simulink model "ssc_aircraft_elec_hybrid"  (R2025a)
settings: Solver=ode23t  StartTime=0.0  StopTime=FlightProfileLength  RelTol=1e-3  AbsTol=1e-3  EnableMultiTasking=on
PreLoadFcn:
  | ssc_aircraft_elec_default_params
PostLoadFcn:
  | warning('off','physmod:common:gl:sli:rtp:InvalidNonValueReference')
  | warning off Simulink:Engine:SortDiscontinuityInAlgLoop
model workspace (MATLAB code in the model file):
  | v0                 = 0; % Initial vehicle speed
  | wheel_radius = 0.15; % Wheel radius
  | k                   = 1e-2; % Motor losses (W/(N*M)^2)
  | t_torque        = 0.02; % Electric motor time constant
  | rpm0             = 2000; % Engine initial speed demand
undefined symbols (not defined in the file): Based, engine_ref_speed, gen_torque_demand, Height, motor_ref_speed
libraries: fl_lib x53, nesl_utility x31, ee_lib x9, ssc_aircraft_elec_lib x2, batteryecm_lib x1, simulink x1, sdl_lib x1, SimscapeFluids_lib x1
(part 2 of 2)

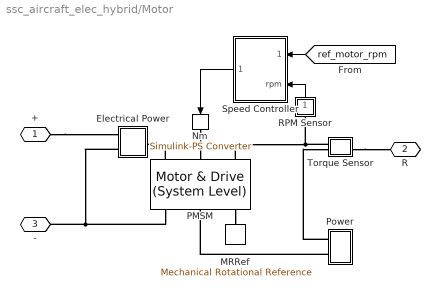
== system ssc_aircraft_elec_hybrid/Motor ==
  Electrical Power : Subsystem
  MRRef : fl_lib/Mechanical/Rotational Elements/Mechanical Rotational Reference
  Nm : nesl_utility/Simulink-PS Converter  PhysicalDomain=network_engine_domain  SubClassName=ps_input  LeftPortType=input  RightPortType=output  PseudoPeriodic=off  Frequencies=[]  NoiseDistribution=none  NoiseParameters=[]  Unit=N*m  AffineConversion=off  FilteringAndDerivatives=zero  SimscapeFilterOrder=1  InputFilterTimeConstant=.001  UdotUserProvided=1
  PMSM : ee_lib/Electromechanical/Motor & Drive (System Level)  torque_speed_param=1  overtorque_param=ee.enum.electromech.overtorque.no  T_t=[ 0.9 0.8 0.7 0 ]*500 N*m  T_t_intermittent=[.36, .32, .28, 0] N*m  T_t_2D=[.09, .09, .09; .08, .08, .08; .07, .07, .07; 0, 0, 0] N*m  T_t_intermittent_2D=[.36, .36, .36; .32, .32, .32; .28, .28, .28; 0, 0, 0] N*m  w_t=[ 0 3.75e+3 7.5e+3 8e+3 ] rpm  vdc_t=[6, 12, 24] V  torque_max=0.1 N*m  power_max=30 W  torque_max_intermittent=0.4 N*m  power_max_intermittent=120 W  time_overtorque=30 s  time_recover=60 s  Tc=0.02 s  EnableSwitch=simscape.enum.onoff.off  losses_param=1  eff=95  w_eff=3.75e+3 rpm  T_eff=400 N*m  Piron=0 W  Pbase=0 W  w_eff_vec=[-8000 -4000 0 4000 8000] rpm  T_eff_vec=[0 0.03 0.06 0.09] N*m  v_eff_vec=[100, 250, 400] V  losses_mat=[1.49 1.67 2.21 3.10; 0.42 0.69 1.14 2.03; 0.06 0.24 0.78 1.68; 0.42 0.69 1.14 2.03; 1.49 1.67 2.21 3.10] W  efficiency_mat=[95 95 95 95; 95 95 95 95; 95 95 95 95; 95 95 95 95; 95 95 95 95]  losses_mat_3D=ones(5, 4, 3) W  efficiency_mat_3D=95 * ones(5, 4, 3)  Res=0 Ohm  J=0 kg*m^2  lam=1e-5 N*m/(rad/s)  speed0=2000 rpm  faulted_specify=off  faulted_priority=None  faulted=0  faulted_nominal_specify=off  faulted_nominal_value=1  faulted_nominal_unit=1  isSwitchedOff_specify=off  isSwitchedOff_priority=None  isSwitchedOff=0  isSwitchedOff_nominal_specify=off  isSwitchedOff_nominal_value=1  isSwitchedOff_nominal_unit=1  torqueLimitContinuous_specify=off  torqueLimitContinuous_priority=None  torqueLimitContinuous=0 N*m  torqueLimitContinuous_nominal_specify=off  torqueLimitContinuous_nominal_value=1  torqueLimitContinuous_nominal_unit=N*m  alpha=3.93e-3 1/K  Tmeas=25 degC  Tmeas2=125 degC  losses_mat_T2=[1.49, 1.74, 2.49, 3.74; .42, .67, 1.42, 2.67; .06, .31, 1.06, 2.31; .42, .67, 1.42, 2.67; 1.49, 1.74, 2.49, 3.74] W  efficiency_mat_T2=[95, 95, 95, 95; 95, 95, 95, 95; 95, 95, 95, 95; 95, 95, 95, 95; 95, 95, 95, 95]  losses_mat_3D_T2=ones(5, 4, 3) W  efficiency_mat_3D_T2=95 * ones(5, 4, 3)  thermal_mass=100 J/K  initial_temperature=25 degC
  Power : Subsystem
  RPM Sensor : Subsystem
      mask Display: disp('w')
  Speed Controller : Subsystem
  Torque Sensor : Subsystem
      mask Display: disp('trq');
  + : PMIOPort  Side=Right
  R : PMIOPort  Port=2  Side=Left
  - : PMIOPort  Port=3  Side=Right
  wires:
  Speed Controller/1(T_ref) -> Nm/1
  [ref_motor_rpm] -> Speed Controller/1(rpm_ref)
  RPM Sensor/1(rpm) -> Speed Controller/2(rpm)
  connections:
  Power/RConn2 -- PMSM/RConn2
  Torque Sensor/RConn1 -- R/RConn1
  Nm/RConn1 -- PMSM/LConn2
  PMSM/LConn3 -- RPM Sensor/LConn1 -- Torque Sensor/LConn1
  Electrical Power/LConn2 -- -/RConn1 -- PMSM/RConn1
  PMSM/LConn1 -- Electrical Power/RConn1
  PMSM/RConn3 -- MRRef/LConn1
  +/RConn1 -- Electrical Power/LConn1
  Power/RConn1 -- Torque Sensor/LConn2

== system ssc_aircraft_elec_hybrid/Routing ==
  M : Inport
  E : Inport  Port=2
  G : Inport  Port=3
  tag scope: ref_engine_speed=global, ref_generator_torque=global, ref_motor_rpm=global
  wires:
  M/1 -> [ref_motor_rpm]  "Ref Motor RPM"
  G/1 -> [ref_generator_torque]
  E/1 -> [ref_engine_speed]

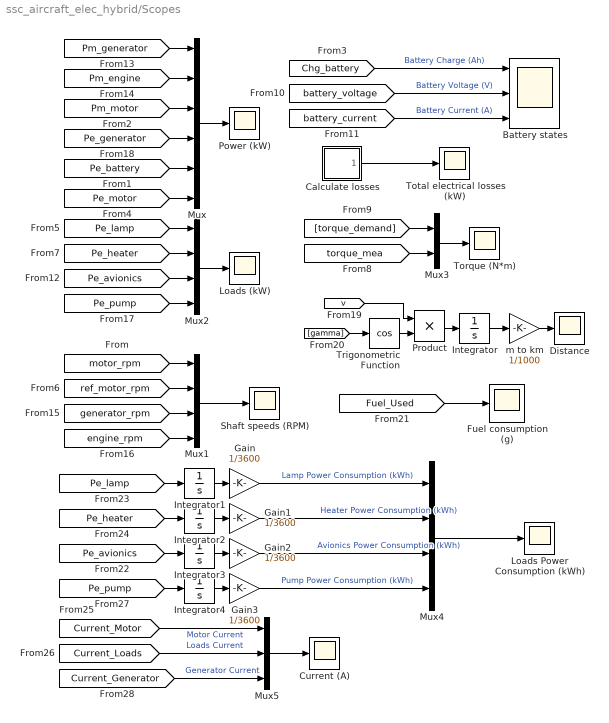
== system ssc_aircraft_elec_hybrid/Scopes ==
  Battery states : Scope  NumInputPorts=3
      settings: ActiveDisplayYMinimum=10  ActiveDisplayYMaximum=110  DataLoggingVariableName=HybridBatteryScopeData
  Calculate losses : Subsystem
  Current (A) : Scope
      settings: TimeSpan=20  ActiveDisplayYMinimum=-113.26291  ActiveDisplayYMaximum=160.64128  DataLoggingMaxPoints=50000  DataLoggingVariableName=HybridCurrentData
  Distance : Scope
      settings: ActiveDisplayYMinimum=-12.7724  ActiveDisplayYMaximum=114.9516  DataLoggingVariableName=Distance  DataLoggingSaveFormat=Array
  Fuel consumption (g) : Scope
      settings: TimeSpan=20  ActiveDisplayYMinimum=-191.16919  ActiveDisplayYMaximum=1720.52275  DataLoggingMaxPoints=50000
  Gain{,1..3} (4 alike) : Gain  Gain=1/3600
  Integrator{,1..4} (5 alike) : Integrator
  Loads (kW) : Scope
      settings: TimeSpan=20  ActiveDisplayYMinimum=-0.2683  ActiveDisplayYMaximum=2.41473  DataLoggingMaxPoints=50000
  Loads Power Consumption (kWh) : Scope
      settings: TimeSpan=20  ActiveDisplayYMinimum=-0.06156  ActiveDisplayYMaximum=0.55406  DataLoggingMaxPoints=50000  DataLoggingVariableName=HybridLoadPowerConsumptionData
  Mux : Mux  Inputs=6
  Mux1 : Mux
  Mux2 : Mux
  Mux3 : Mux  Inputs=2
  Mux4 : Mux
  Mux5 : Mux  Inputs=3
  Power (kW) : Scope
      settings: TimeSpan=20  ActiveDisplayYMinimum=-16.03345  ActiveDisplayYMaximum=35.31999  DataLoggingMaxPoints=50000  DataLoggingVariableName=ScopeData8
  Product : Product
  Shaft speeds (RPM) : Scope
      settings: ActiveDisplayYMinimum=1473.13164  ActiveDisplayYMaximum=2062.04487  DataLoggingMaxPoints=50000
  Torque (N*m) : Scope
      settings: TimeSpan=20  ActiveDisplayYMinimum=-49.62729  ActiveDisplayYMaximum=446.62471  DataLoggingMaxPoints=50000
  Total electrical losses (kW) : Scope
      settings: TimeSpan=20  ActiveDisplayYMinimum=1.3595  ActiveDisplayYMaximum=5.38899  DataLoggingVariableName=ScopeData3
  Trigonometric Function : Trigonometry  Operator=cos
  m to km : Gain  Gain=1/1000
  wires:
  [Chg_battery] -> Battery states/1  "Battery Charge (Ah)"
  Calculate losses/1(Ploss) -> Total electrical losses (kW)/1
  [Pe_battery] -> Mux/5
  [motor_rpm] -> Mux1/1
  Mux1/1 -> Shaft speeds (RPM)/1
  Mux/1 -> Power (kW)/1
  Mux2/1 -> Loads (kW)/1
  [Pe_motor] -> Mux/6
  [Pm_motor] -> Mux/3
  [ref_motor_rpm] -> Mux1/2
  Mux3/1 -> Torque (N*m)/1
  [torque_demand] -> Mux3/1
  [torque_mea] -> Mux3/2
  [battery_voltage] -> Battery states/2  "Battery Voltage (V)"
  [battery_current] -> Battery states/3  "Battery Current (A)"
  [Pe_avionics] -> Mux2/3
  [Pe_lamp] -> Mux2/1
  [Pe_heater] -> Mux2/2
  [Pm_generator] -> Mux/1
  [Pm_engine] -> Mux/2
  [generator_rpm] -> Mux1/3
  [engine_rpm] -> Mux1/4
  [Pe_pump] -> Mux2/4
  [Pe_generator] -> Mux/4
  Integrator/1 -> m to km/1
  [gamma] -> Trigonometric Function/1
  Product/1 -> Integrator/1
  [v] -> Product/1
  Trigonometric Function/1 -> Product/2
  m to km/1 -> Distance/1
  [Fuel_Used] -> Fuel consumption (g)/1
  [Current_Loads] -> Mux5/2  "Loads Current"
  Gain2/1 -> Mux4/3  "Avionics Power Consumption (kWh)"
  [Current_Motor] -> Mux5/1  "Motor Current"
  Gain1/1 -> Mux4/2  "Heater Power Consumption (kWh)"
  Integrator2/1 -> Gain1/1
  Integrator3/1 -> Gain2/1
  Mux5/1 -> Current (A)/1
  [Pe_avionics] -> Integrator3/1
  Gain/1 -> Mux4/1  "Lamp Power Consumption (kWh)"
  [Pe_heater] -> Integrator2/1
  Mux4/1 -> Loads Power Consumption (kWh)/1
  Integrator1/1 -> Gain/1
  [Pe_lamp] -> Integrator1/1
  [Pe_pump] -> Integrator4/1
  Integrator4/1 -> Gain3/1
  Gain3/1 -> Mux4/4  "Pump Power Consumption (kWh)"
  [Current_Generator] -> Mux5/3  "Generator Current"

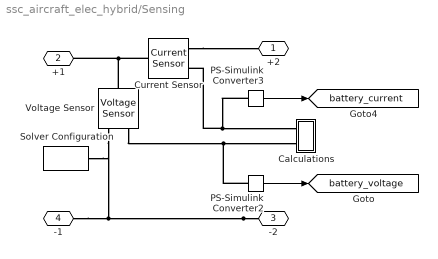
== system ssc_aircraft_elec_hybrid/Sensing ==
  Calculations : Subsystem
  Current Sensor : fl_lib/Electrical/Electrical Sensors/Current Sensor
  PS-Simulink Converter2 : nesl_utility/PS-Simulink Converter  PhysicalDomain=network_engine_domain  SubClassName=ps_output  LeftPortType=input  RightPortType=output  PseudoPeriodic=off  Frequencies=[]  VectorFormat=1-D array  Unit=V  AffineConversion=off
  PS-Simulink Converter3 : nesl_utility/PS-Simulink Converter  PhysicalDomain=network_engine_domain  SubClassName=ps_output  LeftPortType=input  RightPortType=output  PseudoPeriodic=off  Frequencies=[]  VectorFormat=1-D array  Unit=A  AffineConversion=off
  Solver Configuration : nesl_utility/Solver Configuration  PhysicalDomain=network_engine_domain  SubClassName=solver  LeftPortType=input  RightPortType=generic  Tones=[]  Harmonics=[]  SimulateNoise=off  Profile=off  UseLocalSampling=off  EnableSwitchedLinearOptims=on  FrequencyDomain=off  UseCCode=off  RelTol=0.001  AbsTol=1e-06  MinStep=1e-09  ToWorkspace=off  RevertToSquareIcSolve=off  NumHomotopyIterations=100  PhasorMode=off  PhasorModeNumHarmonics=1  ConsistencySolver=NEWTON_FTOL  IndexReductionMethod=DerivativeReplacement  DoDC=off  ResidualTolerance=1e-9  ConsistencyTolSource=GLOBAL  ConsistencyAbsTol=0.001  ConsistencyRelTol=0.001  ConsistencyTolFactor=0.001  UseLocalSolver=off  LocalSolverChoice=NE_BACKWARD_EULER_ADVANCER  ResolveIndetEquations=on  FunctionEvalNumThread=1  LocalSolverSampleTime=0.01  DoFixedCost=off  MaxNonlinIter=3  MaxModeIter=2  ComputeImpulses=off  ImpulseIterations=2  LinearAlgebra=Sparse  LinearAlgebraNumThread=0  EquationFormulation=NE_TIME_EF  DelaysMemoryBudget=1024  AutomaticFiltering=on  FilteringTimeConstant=0.001  PartitionStorageMethod=AS_NEEDED  PartitionMemoryBudget=1024  PartitionMethod=FAST  MultibodyUseLocalSolver=off  MultibodyLocalSolverChoice=ODE1  MultibodyLocalSolverSampleTime=0.001
  Voltage Sensor : fl_lib/Electrical/Electrical Sensors/Voltage Sensor
  +2 : PMIOPort  Side=Right
  +1 : PMIOPort  Port=2  Side=Left
  -2 : PMIOPort  Port=3  Side=Right
  -1 : PMIOPort  Port=4  Side=Left
  tag scope: battery_current=global, battery_voltage=global
  wires:
  PS-Simulink Converter2/1 -> [battery_voltage]
  PS-Simulink Converter3/1 -> [battery_current]
  connections:
  Current Sensor/RConn2 -- +2/RConn1
  PS-Simulink Converter3/LConn1 -- Current Sensor/RConn1 -- Calculations/LConn1
  Voltage Sensor/RConn1 -- PS-Simulink Converter2/LConn1 -- Calculations/LConn2
  Voltage Sensor/LConn1 -- Current Sensor/LConn1 -- +1/RConn1
  -2/RConn1 -- Solver Configuration/RConn1 -- Voltage Sensor/RConn2 -- -1/RConn1

== system ssc_aircraft_elec_hybrid/Avionics/Electrical Power ==
  " W to kW " : Gain  Gain=1/1000
  Current Sensor : fl_lib/Electrical/Electrical Sensors/Current Sensor
  PS Product : fl_lib/Physical Signals/Functions/PS Product
  PS-Simulink Converter3 : nesl_utility/PS-Simulink Converter  PhysicalDomain=network_engine_domain  SubClassName=ps_output  LeftPortType=input  RightPortType=output  PseudoPeriodic=off  Frequencies=[]  VectorFormat=1-D array  Unit=W  AffineConversion=off
  Voltage Sensor : fl_lib/Electrical/Electrical Sensors/Voltage Sensor
  + : PMIOPort  Side=Left
  - : PMIOPort  Port=2  Side=Right
  0v : PMIOPort  Port=3  Side=Left
  tag scope: Pe_avionics=global
  wires:
  PS-Simulink Converter3/1 -> " W to kW "/1
  " W to kW "/1 -> [Pe_avionics]  "Avionics Power (kW)"
  connections:
  Current Sensor/RConn1 -- PS Product/LConn1
  -/RConn1 -- Current Sensor/RConn2 -- Voltage Sensor/LConn1
  Current Sensor/LConn1 -- +/RConn1
  0v/RConn1 -- Voltage Sensor/RConn2
  Voltage Sensor/RConn1 -- PS Product/LConn2
  PS Product/RConn1 -- PS-Simulink Converter3/LConn1

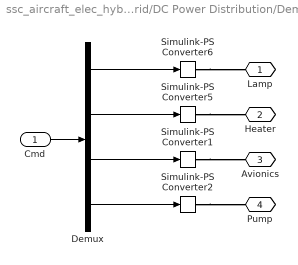
== system ssc_aircraft_elec_hybrid/DC Power Distribution/Demux ==
  Cmd : Inport
  Demux : Demux
  Simulink-PS Converter{1..2,5..6} (4 alike) : nesl_utility/Simulink-PS Converter  PhysicalDomain=network_engine_domain  SubClassName=ps_input  LeftPortType=input  RightPortType=output  PseudoPeriodic=off  Frequencies=[]  NoiseDistribution=none  NoiseParameters=[]  Unit=1  AffineConversion=off  FilteringAndDerivatives=zero  SimscapeFilterOrder=1  InputFilterTimeConstant=0.001  UdotUserProvided=1
  Lamp : PMIOPort  Side=Right
  Heater : PMIOPort  Port=2  Side=Right
  Avionics : PMIOPort  Port=3  Side=Right
  Pump : PMIOPort  Port=4  Side=Right
  wires:
  Demux/2 -> Simulink-PS Converter5/1
  Demux/3 -> Simulink-PS Converter1/1
  Demux/4 -> Simulink-PS Converter2/1
  Cmd/1 -> Demux/1
  Demux/1 -> Simulink-PS Converter6/1
  connections:
  Simulink-PS Converter6/RConn1 -- Lamp/RConn1
  Simulink-PS Converter5/RConn1 -- Heater/RConn1
  Simulink-PS Converter2/RConn1 -- Pump/RConn1
  Simulink-PS Converter1/RConn1 -- Avionics/RConn1

== system ssc_aircraft_elec_hybrid/DC Power Distribution/Sensing Current ==
  Current Sensor : fl_lib/Electrical/Electrical Sensors/Current Sensor
  PS-Simulink Converter1 : nesl_utility/PS-Simulink Converter  PhysicalDomain=network_engine_domain  SubClassName=ps_output  LeftPortType=input  RightPortType=output  PseudoPeriodic=off  Frequencies=[]  VectorFormat=1-D array  Unit=1  AffineConversion=off
  + : PMIOPort  Side=Left
  - : PMIOPort  Port=2  Side=Right
  tag scope: Current_Loads=global
  wires:
  PS-Simulink Converter1/1 -> [Current_Loads]
  connections:
  Current Sensor/RConn2 -- -/RConn1
  Current Sensor/LConn1 -- +/RConn1
  Current Sensor/RConn1 -- PS-Simulink Converter1/LConn1

== system ssc_aircraft_elec_hybrid/Engine/Engine Management ==
  rpm_dem : Inport
  rpm : Inport  Port=2
  Kp : Gain  Gain=1e-3  SaturateOnIntegerOverflow=on  OutDataTypeStr=Inherit: Same as input  ParamDataTypeStr=Inherit: Same as input
  Sum2 : Sum  Inputs=+-|  InputSameDT=on  SaturateOnIntegerOverflow=on  OutDataTypeStr=Inherit: Same as first input
  "[0,1]" : Saturate  UpperLimit=1  LowerLimit=0
  T : Outport  VectorParamsAs1DForOutWhenUnconnected=off
  wires:
  rpm/1 -> Sum2/2
  rpm_dem/1 -> Sum2/1
  Sum2/1 -> Kp/1
  Kp/1 -> "[0,1]"/1
  "[0,1]"/1 -> T/1

== system ssc_aircraft_elec_hybrid/Engine/RPM Sensor ==
  Ideal Rotational Motion Sensor : fl_lib/Mechanical/Mechanical Sensors/Ideal Rotational Motion Sensor  reference=foundation.enum.MeasurementReference.difference  acceleration_port=false  velocity_port=true  position_port=true  wrap_angle=simscape.enum.onoff.off  offset=0 rad
  MRR : fl_lib/Mechanical/Rotational Elements/Mechanical Rotational Reference
  PS2S : nesl_utility/PS-Simulink Converter  PhysicalDomain=network_engine_domain  SubClassName=ps_output  LeftPortType=input  RightPortType=output  PseudoPeriodic=off  Frequencies=[]  VectorFormat=1-D array  Unit=rpm  AffineConversion=off
  Sensor dynamics : TransferFcn  Denominator=[0.01 1]
  F : PMIOPort  Side=Left
  rpm : Outport  VectorParamsAs1DForOutWhenUnconnected=off
  tag scope: engine_rpm=global
  wires:
  PS2S/1 -> Sensor dynamics/1, [engine_rpm]  "Engine RPM"
  Sensor dynamics/1 -> rpm/1
  connections:
  F/RConn1 -- Ideal Rotational Motion Sensor/LConn1
  Ideal Rotational Motion Sensor/RConn2 -- PS2S/LConn1
  MRR/LConn1 -- Ideal Rotational Motion Sensor/RConn1

== system ssc_aircraft_elec_hybrid/Engine/Sensor Fuel ==
  Integrator : Integrator
  PS2S2 : nesl_utility/PS-Simulink Converter  PhysicalDomain=network_engine_domain  SubClassName=ps_output  LeftPortType=input  RightPortType=output  PseudoPeriodic=off  Frequencies=[]  VectorFormat=1-D array  Unit=g/s  AffineConversion=off
  FC : PMIOPort  Side=Left
  tag scope: Fuel_Used=global
  wires:
  PS2S2/1 -> Integrator/1
  Integrator/1 -> [Fuel_Used]
  connections:
  FC/RConn1 -- PS2S2/LConn1

== system ssc_aircraft_elec_hybrid/Engine/Sensor Power ==
  PS2S1 : nesl_utility/PS-Simulink Converter  PhysicalDomain=network_engine_domain  SubClassName=ps_output  LeftPortType=input  RightPortType=output  PseudoPeriodic=off  Frequencies=[]  VectorFormat=1-D array  Unit=kW  AffineConversion=off
  P : PMIOPort  Side=Left
  tag scope: Pm_engine=global
  wires:
  PS2S1/1 -> [Pm_engine]  "Engine Mechanical Power"
  connections:
  P/RConn1 -- PS2S1/LConn1

== system ssc_aircraft_elec_hybrid/Fuel Pump/Electrical Power ==
  " W to kW " : Gain  Gain=1/1000
  Current Sensor : fl_lib/Electrical/Electrical Sensors/Current Sensor
  PS Product : fl_lib/Physical Signals/Functions/PS Product
  PS-Simulink Converter3 : nesl_utility/PS-Simulink Converter  PhysicalDomain=network_engine_domain  SubClassName=ps_output  LeftPortType=input  RightPortType=output  PseudoPeriodic=off  Frequencies=[]  VectorFormat=1-D array  Unit=W  AffineConversion=off
  Voltage Sensor : fl_lib/Electrical/Electrical Sensors/Voltage Sensor
  + : PMIOPort  Side=Left
  - : PMIOPort  Port=2  Side=Right
  0v : PMIOPort  Port=3  Side=Left
  tag scope: Pe_pump=global
  wires:
  " W to kW "/1 -> [Pe_pump]  "Pump Power (kW)"
  PS-Simulink Converter3/1 -> " W to kW "/1
  connections:
  PS Product/RConn1 -- PS-Simulink Converter3/LConn1
  Voltage Sensor/RConn1 -- PS Product/LConn2
  0v/RConn1 -- Voltage Sensor/RConn2
  Current Sensor/LConn1 -- +/RConn1
  Voltage Sensor/LConn1 -- Current Sensor/RConn2 -- -/RConn1
  Current Sensor/RConn1 -- PS Product/LConn1

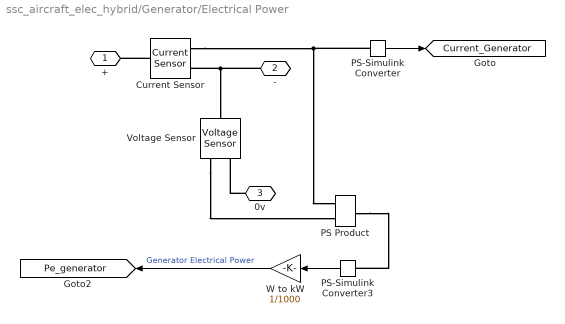
== system ssc_aircraft_elec_hybrid/Generator/Electrical Power ==
  " W to kW " : Gain  Gain=1/1000
  Current Sensor : fl_lib/Electrical/Electrical Sensors/Current Sensor
  PS Product : fl_lib/Physical Signals/Functions/PS Product
  PS-Simulink Converter : nesl_utility/PS-Simulink Converter  PhysicalDomain=network_engine_domain  SubClassName=ps_output  LeftPortType=input  RightPortType=output  PseudoPeriodic=off  Frequencies=[]  VectorFormat=1-D array  Unit=1  AffineConversion=off
  PS-Simulink Converter3 : nesl_utility/PS-Simulink Converter  PhysicalDomain=network_engine_domain  SubClassName=ps_output  LeftPortType=input  RightPortType=output  PseudoPeriodic=off  Frequencies=[]  VectorFormat=1-D array  Unit=W  AffineConversion=off
  Voltage Sensor : fl_lib/Electrical/Electrical Sensors/Voltage Sensor
  + : PMIOPort  Side=Left
  - : PMIOPort  Port=2  Side=Right
  0v : PMIOPort  Port=3  Side=Left
  tag scope: Current_Generator=global, Pe_generator=global
  wires:
  PS-Simulink Converter3/1 -> " W to kW "/1
  " W to kW "/1 -> [Pe_generator]  "Generator Electrical Power"
  PS-Simulink Converter/1 -> [Current_Generator]
  connections:
  Current Sensor/RConn1 -- PS-Simulink Converter/LConn1 -- PS Product/LConn1
  -/RConn1 -- Voltage Sensor/LConn1 -- Current Sensor/RConn2
  Current Sensor/LConn1 -- +/RConn1
  0v/RConn1 -- Voltage Sensor/RConn2
  Voltage Sensor/RConn1 -- PS Product/LConn2
  PS Product/RConn1 -- PS-Simulink Converter3/LConn1

== system ssc_aircraft_elec_hybrid/Generator/Power ==
  " W to kW " : Gain  Gain=1/1000
  PS Product : fl_lib/Physical Signals/Functions/PS Product
  PS-Simulink Converter3 : nesl_utility/PS-Simulink Converter  PhysicalDomain=network_engine_domain  SubClassName=ps_output  LeftPortType=input  RightPortType=output  PseudoPeriodic=off  Frequencies=[]  VectorFormat=1-D array  Unit=W  AffineConversion=off
  trq : PMIOPort  Side=Right
  w : PMIOPort  Port=2  Side=Right
  tag scope: Pm_generator=global
  wires:
  PS-Simulink Converter3/1 -> " W to kW "/1
  " W to kW "/1 -> [Pm_generator]  "Generator Mechanical Power"
  connections:
  PS Product/RConn1 -- PS-Simulink Converter3/LConn1
  PS Product/LConn2 -- w/RConn1
  PS Product/LConn1 -- trq/RConn1

== system ssc_aircraft_elec_hybrid/Generator/RPM Sensor ==
  MRRef : fl_lib/Mechanical/Rotational Elements/Mechanical Rotational Reference
  Motion Sensor : fl_lib/Mechanical/Mechanical Sensors/Ideal Rotational Motion Sensor  reference=foundation.enum.MeasurementReference.difference  acceleration_port=false  velocity_port=true  position_port=true  wrap_angle=simscape.enum.onoff.off  offset=0 rad
  PS-Simulink Converter 2 : nesl_utility/PS-Simulink Converter  PhysicalDomain=network_engine_domain  SubClassName=ps_output  LeftPortType=input  RightPortType=output  PseudoPeriodic=off  Frequencies=[]  VectorFormat=1-D array  Unit=rpm  AffineConversion=off
  R : PMIOPort  Side=Left
  tag scope: generator_rpm=global
  wires:
  PS-Simulink Converter 2/1 -> [generator_rpm]  "Generator RPM"
  connections:
  R/RConn1 -- Motion Sensor/LConn1
  Motion Sensor/RConn1 -- MRRef/LConn1
  Motion Sensor/RConn2 -- PS-Simulink Converter 2/LConn1

== system ssc_aircraft_elec_hybrid/Generator/Torque Sensor ==
  Torque Sensor : fl_lib/Mechanical/Mechanical Sensors/Ideal Torque Sensor
  C : PMIOPort  Side=Right
  R : PMIOPort  Port=2  Side=Left
  trq : PMIOPort  Port=3  Side=Left
  connections:
  Torque Sensor/RConn1 -- C/RConn1
  trq/RConn1 -- Torque Sensor/RConn2
  R/RConn1 -- Torque Sensor/LConn1

== system ssc_aircraft_elec_hybrid/Heater/Electrical Power ==
  " W to kW " : Gain  Gain=1/1000
  Current Sensor : fl_lib/Electrical/Electrical Sensors/Current Sensor
  PS Product : fl_lib/Physical Signals/Functions/PS Product
  PS-Simulink Converter3 : nesl_utility/PS-Simulink Converter  PhysicalDomain=network_engine_domain  SubClassName=ps_output  LeftPortType=input  RightPortType=output  PseudoPeriodic=off  Frequencies=[]  VectorFormat=1-D array  Unit=W  AffineConversion=off
  Voltage Sensor : fl_lib/Electrical/Electrical Sensors/Voltage Sensor
  + : PMIOPort  Side=Left
  - : PMIOPort  Port=2  Side=Right
  0v : PMIOPort  Port=3  Side=Left
  tag scope: Pe_heater=global
  wires:
  " W to kW "/1 -> [Pe_heater]  "Heater Power (kW)"
  PS-Simulink Converter3/1 -> " W to kW "/1
  connections:
  PS Product/RConn1 -- PS-Simulink Converter3/LConn1
  Voltage Sensor/RConn1 -- PS Product/LConn2
  0v/RConn1 -- Voltage Sensor/RConn2
  Current Sensor/LConn1 -- +/RConn1
  Voltage Sensor/LConn1 -- Current Sensor/RConn2 -- -/RConn1
  Current Sensor/RConn1 -- PS Product/LConn1

== system ssc_aircraft_elec_hybrid/Lamp/Electrical Power ==
  " W to kW " : Gain  Gain=1/1000
  Current Sensor : fl_lib/Electrical/Electrical Sensors/Current Sensor
  PS Product : fl_lib/Physical Signals/Functions/PS Product
  PS-Simulink Converter3 : nesl_utility/PS-Simulink Converter  PhysicalDomain=network_engine_domain  SubClassName=ps_output  LeftPortType=input  RightPortType=output  PseudoPeriodic=off  Frequencies=[]  VectorFormat=1-D array  Unit=W  AffineConversion=off
  Voltage Sensor : fl_lib/Electrical/Electrical Sensors/Voltage Sensor
  + : PMIOPort  Side=Left
  - : PMIOPort  Port=2  Side=Right
  0v : PMIOPort  Port=3  Side=Left
  tag scope: Pe_lamp=global
  wires:
  " W to kW "/1 -> [Pe_lamp]  "Lamp Power (kW)"
  PS-Simulink Converter3/1 -> " W to kW "/1
  connections:
  PS Product/RConn1 -- PS-Simulink Converter3/LConn1
  Voltage Sensor/RConn1 -- PS Product/LConn2
  0v/RConn1 -- Voltage Sensor/RConn2
  Current Sensor/LConn1 -- +/RConn1
  Voltage Sensor/LConn1 -- Current Sensor/RConn2 -- -/RConn1
  Current Sensor/RConn1 -- PS Product/LConn1

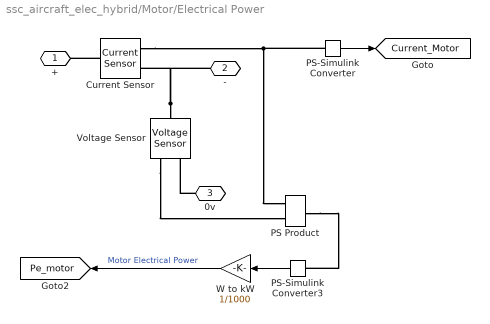
== system ssc_aircraft_elec_hybrid/Motor/Electrical Power ==
  " W to kW " : Gain  Gain=1/1000
  Current Sensor : fl_lib/Electrical/Electrical Sensors/Current Sensor
  PS Product : fl_lib/Physical Signals/Functions/PS Product
  PS-Simulink Converter : nesl_utility/PS-Simulink Converter  PhysicalDomain=network_engine_domain  SubClassName=ps_output  LeftPortType=input  RightPortType=output  PseudoPeriodic=off  Frequencies=[]  VectorFormat=1-D array  Unit=1  AffineConversion=off
  PS-Simulink Converter3 : nesl_utility/PS-Simulink Converter  PhysicalDomain=network_engine_domain  SubClassName=ps_output  LeftPortType=input  RightPortType=output  PseudoPeriodic=off  Frequencies=[]  VectorFormat=1-D array  Unit=W  AffineConversion=off
  Voltage Sensor : fl_lib/Electrical/Electrical Sensors/Voltage Sensor
  + : PMIOPort  Side=Left
  - : PMIOPort  Port=2  Side=Right
  0v : PMIOPort  Port=3  Side=Left
  tag scope: Current_Motor=global, Pe_motor=global
  wires:
  " W to kW "/1 -> [Pe_motor]  "Motor Electrical Power"
  PS-Simulink Converter3/1 -> " W to kW "/1
  PS-Simulink Converter/1 -> [Current_Motor]
  connections:
  PS Product/RConn1 -- PS-Simulink Converter3/LConn1
  Voltage Sensor/RConn1 -- PS Product/LConn2
  0v/RConn1 -- Voltage Sensor/RConn2
  Current Sensor/LConn1 -- +/RConn1
  Voltage Sensor/LConn1 -- Current Sensor/RConn2 -- -/RConn1
  Current Sensor/RConn1 -- PS-Simulink Converter/LConn1 -- PS Product/LConn1

== system ssc_aircraft_elec_hybrid/Motor/Power ==
  " W to kW " : Gain  Gain=1/1000
  PS Product : fl_lib/Physical Signals/Functions/PS Product
  PS-Simulink Converter3 : nesl_utility/PS-Simulink Converter  PhysicalDomain=network_engine_domain  SubClassName=ps_output  LeftPortType=input  RightPortType=output  PseudoPeriodic=off  Frequencies=[]  VectorFormat=1-D array  Unit=W  AffineConversion=off
  trq : PMIOPort  Side=Right
  w : PMIOPort  Port=2  Side=Right
  tag scope: Pm_motor=global
  wires:
  " W to kW "/1 -> [Pm_motor]  "Motor Mechanical Power"
  PS-Simulink Converter3/1 -> " W to kW "/1
  connections:
  PS Product/LConn1 -- trq/RConn1
  PS Product/LConn2 -- w/RConn1
  PS Product/RConn1 -- PS-Simulink Converter3/LConn1

== system ssc_aircraft_elec_hybrid/Motor/RPM Sensor ==
  MRRef : fl_lib/Mechanical/Rotational Elements/Mechanical Rotational Reference
  Motion Sensor : fl_lib/Mechanical/Mechanical Sensors/Ideal Rotational Motion Sensor  reference=foundation.enum.MeasurementReference.difference  acceleration_port=false  velocity_port=true  position_port=true  wrap_angle=simscape.enum.onoff.off  offset=0 rad
  PS-Simulink Converter 2 : nesl_utility/PS-Simulink Converter  PhysicalDomain=network_engine_domain  SubClassName=ps_output  LeftPortType=input  RightPortType=output  PseudoPeriodic=off  Frequencies=[]  VectorFormat=1-D array  Unit=rpm  AffineConversion=off
  R : PMIOPort  Side=Left
  rpm : Outport  VectorParamsAs1DForOutWhenUnconnected=off
  tag scope: motor_rpm=global
  wires:
  PS-Simulink Converter 2/1 -> [motor_rpm], rpm/1  "Motor RPM"
  connections:
  R/RConn1 -- Motion Sensor/LConn1
  Motion Sensor/RConn1 -- MRRef/LConn1
  Motion Sensor/RConn2 -- PS-Simulink Converter 2/LConn1

== system ssc_aircraft_elec_hybrid/Motor/Speed Controller ==
  rpm_ref : Inport
  rpm : Inport  Port=2
  20Hz Lowpass Filter : TransferFcn  Commented=through  Denominator=[1/(2*pi*20) 1]
  Ki : Gain  Gain=60
  Kp : Gain  Gain=60
  Limits [-40,40] : Integrator  LimitOutput=on  UpperSaturationLimit=40  LowerSaturationLimit=-40
  Sum : Sum  Inputs=-+|
  Sum1 : Sum  Inputs=++|
  "[-40,40]" : Saturate  UpperLimit=400  LowerLimit=-400
  T_ref : Outport  VectorParamsAs1DForOutWhenUnconnected=off
  wires:
  "[-40,40]"/1 -> T_ref/1
  20Hz Lowpass Filter/1 -> Sum/1
  Limits [-40,40]/1 -> Sum1/1
  Kp/1 -> Sum1/2
  Ki/1 -> Limits [-40,40]/1
  Sum/1 -> Kp/1, Ki/1
  Sum1/1 -> "[-40,40]"/1
  rpm/1 -> 20Hz Lowpass Filter/1
  rpm_ref/1 -> Sum/2

== system ssc_aircraft_elec_hybrid/Motor/Torque Sensor ==
  PS-Simulink Converter : nesl_utility/PS-Simulink Converter  PhysicalDomain=network_engine_domain  SubClassName=ps_output  LeftPortType=input  RightPortType=output  PseudoPeriodic=off  Frequencies=[]  VectorFormat=1-D array  Unit=1  AffineConversion=off
  Torque Sensor : fl_lib/Mechanical/Mechanical Sensors/Ideal Torque Sensor
  C : PMIOPort  Side=Right
  R : PMIOPort  Port=2  Side=Left
  trq : PMIOPort  Port=3  Side=Left
  tag scope: torque_mea=global
  wires:
  PS-Simulink Converter/1 -> [torque_mea]  "Measured Torque"
  connections:
  Torque Sensor/RConn2 -- trq/RConn1 -- PS-Simulink Converter/LConn1
  Torque Sensor/RConn1 -- C/RConn1
  Torque Sensor/LConn1 -- R/RConn1

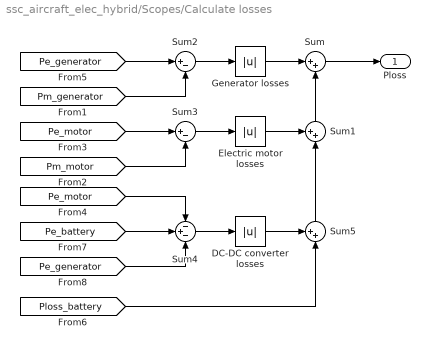
== system ssc_aircraft_elec_hybrid/Scopes/Calculate losses ==
  " Electric motor losses" : Abs
  DC-DC converter losses : Abs
  Generator losses : Abs
  Sum : Sum  Inputs=|++
  Sum1 : Sum  Inputs=++|
  Sum2 : Sum  Inputs=|+-
  Sum3 : Sum  Inputs=|+-
  Sum4 : Sum  Inputs=-+-
  Sum5 : Sum  Inputs=++|
  Ploss : Outport  VectorParamsAs1DForOutWhenUnconnected=off
  wires:
  [Ploss_battery] -> Sum5/2
  DC-DC converter losses/1 -> Sum5/1
  " Electric motor losses"/1 -> Sum1/1
  [Pe_generator] -> Sum4/3
  [Pe_motor] -> Sum4/1
  [Pe_battery] -> Sum4/2
  Sum5/1 -> Sum1/2
  Sum4/1 -> DC-DC converter losses/1
  Sum3/1 -> " Electric motor losses"/1
  [Pm_motor] -> Sum3/2
  [Pe_motor] -> Sum3/1
  Generator losses/1 -> Sum/1
  Sum2/1 -> Generator losses/1
  [Pm_generator] -> Sum2/2
  [Pe_generator] -> Sum2/1
  Sum/1 -> Ploss/1
  Sum1/1 -> Sum/2

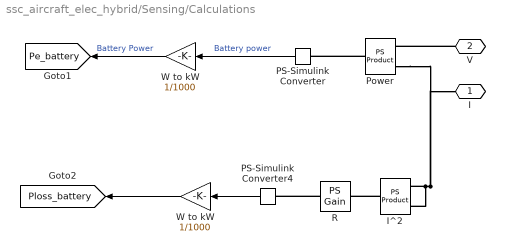
== system ssc_aircraft_elec_hybrid/Sensing/Calculations ==
  " W to kW " : Gain  Gain=1/1000
  I^2 : fl_lib/Physical Signals/Functions/PS Product
  PS-Simulink Converter : nesl_utility/PS-Simulink Converter  PhysicalDomain=network_engine_domain  SubClassName=ps_output  LeftPortType=input  RightPortType=output  PseudoPeriodic=off  Frequencies=[]  VectorFormat=1-D array  Unit=W  AffineConversion=off
  PS-Simulink Converter4 : nesl_utility/PS-Simulink Converter  PhysicalDomain=network_engine_domain  SubClassName=ps_output  LeftPortType=input  RightPortType=output  PseudoPeriodic=off  Frequencies=[]  VectorFormat=1-D array  Unit=W  AffineConversion=off
  Power : fl_lib/Physical Signals/Functions/PS Product
  R : fl_lib/Physical Signals/Functions/PS Gain  gain=0.05 Ohm
  W to kW : Gain  Gain=1/1000
  I : PMIOPort  Side=Left
  V : PMIOPort  Port=2  Side=Left
  tag scope: Pe_battery=global, Ploss_battery=global
  wires:
  " W to kW "/1 -> [Ploss_battery]
  PS-Simulink Converter4/1 -> " W to kW "/1
  W to kW/1 -> [Pe_battery]  "Battery Power"
  PS-Simulink Converter/1 -> W to kW/1  "Battery power"
  connections:
  R/RConn1 -- PS-Simulink Converter4/LConn1
  I^2/RConn1 -- R/LConn1
  I^2/LConn1 -- I^2/LConn2 -- I/RConn1 -- Power/LConn2
  V/RConn1 -- Power/LConn1
  Power/RConn1 -- PS-Simulink Converter/LConn1
